simulink model "mdl_VD_st2dofTireForcesLinear_R2025b_SLX"  (R2025b)
settings: Solver=ode4  StartTime=startTime  StopTime=endTime  FixedStep=deltaT  MaxStep=deltaT  RelTol=1e-3  EnableMultiTasking=on
undefined symbols (not defined in the file): Caf, Car
settings Model: Creator=snb10  LastModifiedBy=snb10
settings SolverCC: AlgebraicLoopSolver=TrustRegion
settings DataIOCC: LimitDataPoints=on  SaveFormat=Array  SignalLoggingSaveFormat=ModelDataLogs  SaveOutput=off  SignalLogging=off  DSMLogging=off  SaveTime=off  SignalLoggingName=sigsOut
settings OptimizationCC: InitFltsAndDblsToZero=on  LifeSpan=inf
settings DebuggingCC: SaveWithParameterizedLinksMsg=none  UnderspecifiedInitializationDetection=Classic  MergeDetectMultiDrivingBlocksExec=none  SignalResolutionControl=TryResolveAllWithWarning  MultiTaskDSMMsg=warning  MultiTaskCondExecSysMsg=none  FcnCallInpInsideContextMsg=warning  UnconnectedInputMsg=warning  UnconnectedOutputMsg=warning  UnconnectedLineMsg=warning  StateNameClashWarn=warning  SFUnexpectedBacktrackingDiag=warning  SFNoUnconditionalDefaultTransitionDiag=warning  SFExecutionAtInitializationDiag=none  ArithmeticOperatorsInVariantConditions=warning
settings HardwareCC: ProdBitPerPointer=32.0  ProdBitPerSizeT=32.0  ProdBitPerPtrDiffT=32.0  ProdLargestAtomicFloat=None  ProdIntDivRoundTo=Undefined  ProdEndianess=Unspecified  ProdWordSize=32.0  ProdHWDeviceType=32-bit Generic  TargetUnknown=on
settings ModelReferenceCC: EnableRefExpFcnMdlSchedulingChecks=on  PropagateSignalLabelsOutOfModel=off
settings SFSimCC: SimUseLocalCustomCode=off  CustomCodeUndefinedFunction=UseInterfaceOnly
settings RTWCC: RTWUseLocalCustomCode=off  GPUComputeCapability=3.5  DLArmComputeVersion=19.05
settings CodeAppCC: StateflowObjectComments=on
settings GRTTargetCC: TargetFcnLib=ansi_tfl_tmw.mat  TargetLangStandard=C89/C90 (ANSI)  CombineOutputUpdateFcns=off  GRTInterface=on
settings ConfigComp: CovMetricSettings=dw  CovSaveCumulativeToWorkspaceVar=on  CovSaveSingleToWorkspaceVar=on  CovExternalEMLEnable=off

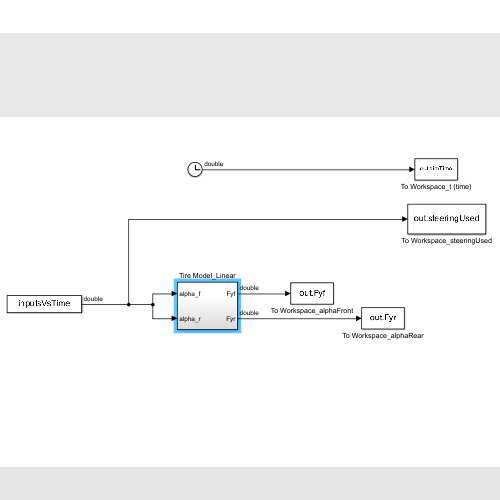
[thumbnail: Simulink's stored preview of the top-level diagram]
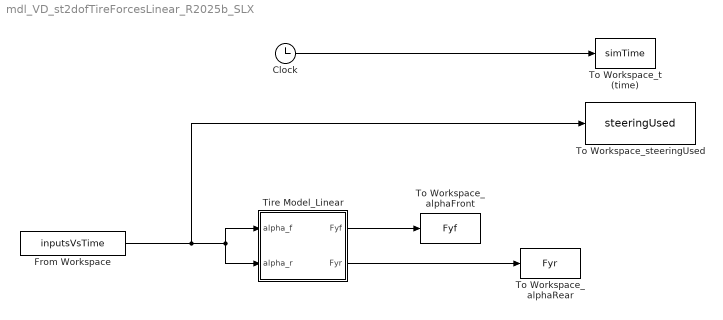
== system mdl_VD_st2dofTireForcesLinear_R2025b_SLX ==
  Clock : Clock
  From Workspace : FromWorkspace  VariableName=inputsVsTime  OutDataTypeStr=double  SampleTime=.01  OutputAfterFinalValue=Holding final value
  Tire Model_Linear : Subsystem
  To Workspace_alphaFront : ToWorkspace  VariableName=Fyf  SampleTime=.01
  To Workspace_alphaRear : ToWorkspace  VariableName=Fyr  SampleTime=.01
  To Workspace_steeringUsed : ToWorkspace  VariableName=steeringUsed  SampleTime=.01
  To Workspace_t (time) : ToWorkspace  VariableName=simTime  SampleTime=.01
  wires:
  Clock/1 -> To Workspace_t (time)/1
  From Workspace/1 -> Tire Model_Linear/1(alpha_f), Tire Model_Linear/2(alpha_r), To Workspace_steeringUsed/1
  Tire Model_Linear/1(Fyf) -> To Workspace_alphaFront/1
  Tire Model_Linear/2(Fyr) -> To Workspace_alphaRear/1

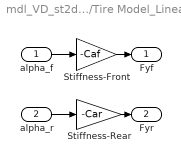
== system mdl_VD_st2dofTireForcesLinear_R2025b_SLX/Tire Model_Linear ==
  alpha_f : Inport
  alpha_r : Inport  Port=2
  Stiffness-Front : Gain  Gain=-Caf
  Stiffness-Rear : Gain  Gain=-Car
  Fyf : Outport
  Fyr : Outport  Port=2
  wires:
  alpha_f/1 -> Stiffness-Front/1
  Stiffness-Front/1 -> Fyf/1
  alpha_r/1 -> Stiffness-Rear/1
  Stiffness-Rear/1 -> Fyr/1
